simulink model "library"  (R2026b)
settings: Solver=VariableStepAuto
undefined symbols (not defined in the file or in its folder): A_mis_sT, D_b, D_p, D_w, DiscIntNeverNeededParam, fi_acc, fixedStep, k_scale, max_slew_rate, N_B, P_max, P_vec, psi_acc, R_E, sT_bias, theta_acc, Ts
libraries: $bdroot x15, matrix_library x4, simulink x2, backup x1
settings Model: Creator=laythe  LastModifiedBy=laythe

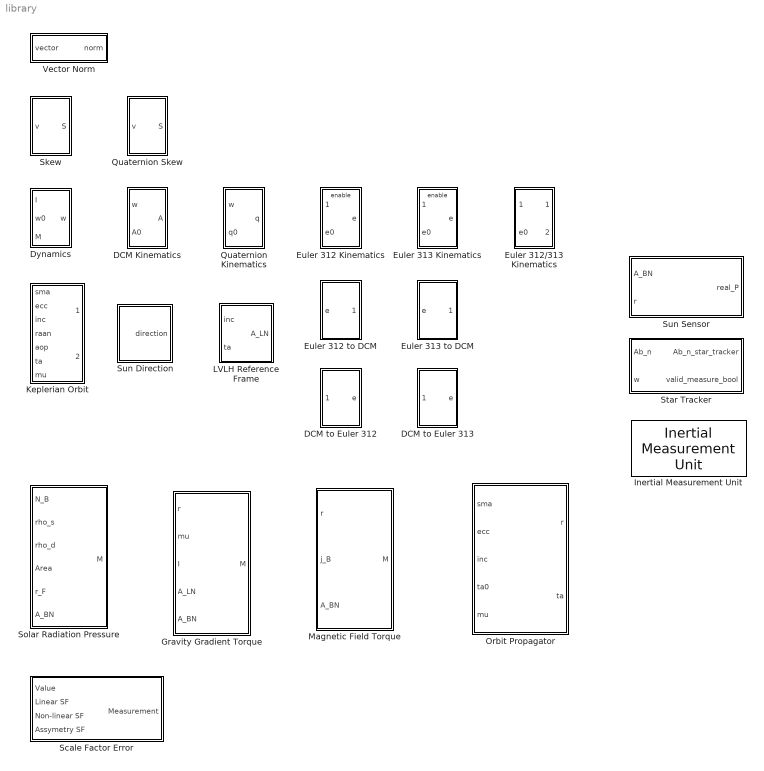
== system library ==
  DCM Kinematics : Subsystem
  DCM to Euler 312 : Subsystem
  DCM to Euler 313 : Subsystem
  Dynamics : Subsystem
  Euler 312 Kinematics : Subsystem
  Euler 312 to DCM : Subsystem
  Euler 312/313 Kinematics : Subsystem
  Euler 313 Kinematics : Subsystem
  Euler 313 to DCM : Subsystem
  Gravity Gradient Torque : Subsystem
  Inertial Measurement Unit : backup/Inertial Measurement Unit  SystemSampleTime=-1  VariantActivationTime=update diagram  EmptyChoice=off  PassThrough=off  PassThroughVariantControl=(default)  EmptyChoiceVariantControl=(default)  AllowFlexibleInterface=on  Latency=0  AutoFrameSizeCalculation=off
  Keplerian Orbit : Subsystem
  LVLH Reference Frame : Subsystem  Description=Inputs: theta_rad (true anomaly), inclination_rad; scalar angles in radians. Output: 3x3 A_LN = Rz_passive(theta)*Rx_passive(i). Maps inertial columns to radial/transverse/normal axes for RAAN=argument of periapsis=0. Exactly the supplied matrix product. No workspace variables.
  Magnetic Field Torque : Subsystem
  Orbit Propagator : Subsystem
  Quaternion Kinematics : Subsystem
  Quaternion Skew : Subsystem
  Scale Factor Error : Subsystem
  Skew : Subsystem
  Solar Radiation Pressure : Subsystem
  Star Tracker : Subsystem
  Sun Direction : Subsystem
  Sun Sensor : Subsystem
  Vector Norm : Subsystem

== system library/DCM Kinematics ==
  w : Inport
  A0 : Inport  Port=2
  Gain : Gain  Gain=-1
  Gain1 : Gain  Gain=1.5
  Gain2 : Gain  Gain=0.5
  Integrator : Integrator  InitialConditionSource=external
  Matrix Multiply : Product  Multiplication=Matrix(*)
  Matrix Multiply1 : Product  Multiplication=Matrix(*)
  Matrix Multiply2 : Product  Multiplication=Matrix(*)
  Skew : $bdroot/Skew  SystemSampleTime=-1  VariantActivationTime=update diagram  EmptyChoice=off  PassThrough=off  PassThroughVariantControl=(default)  EmptyChoiceVariantControl=(default)  AllowFlexibleInterface=on  Latency=0  AutoFrameSizeCalculation=off
  Subtract : Sum  Inputs=+-
  Transpose : Math  Operator=transpose
  A : Outport
  wires:
  Matrix Multiply/1 -> Integrator/1
  A0/1 -> Integrator/2
  Gain/1 -> Matrix Multiply/1
  Skew/1 -> Gain/1
  w/1 -> Skew/1
  Subtract/1 -> Matrix Multiply/2, A/1
  Integrator/1 -> Matrix Multiply2/2, Transpose/1, Matrix Multiply1/1, Gain1/1
  Transpose/1 -> Matrix Multiply1/2
  Matrix Multiply1/1 -> Matrix Multiply2/1
  Matrix Multiply2/1 -> Gain2/1
  Gain1/1 -> Subtract/1
  Gain2/1 -> Subtract/2

== system library/DCM to Euler 312 ==
  DCM : Inport
  Asin : Trigonometry  Operator=asin
  Atan1 : Trigonometry  Operator=atan2
  Atan2 : Trigonometry  Operator=atan2
  Demux : Demux  Outputs=9
  Gain : Gain  Gain=-1
  Gain1 : Gain  Gain=-1
  Mux : Mux  Inputs=3
  Reshape : Reshape  OutputDimensionality=Customize  OutputDimensions=[9,1]
  e : Outport
  wires:
  Demux/8 -> Asin/1
  Asin/1 -> Mux/2
  Atan2/1 -> Mux/1
  Atan1/1 -> Mux/3
  Demux/5 -> Atan2/2
  Demux/9 -> Atan1/2
  Gain/1 -> Atan2/1
  Demux/2 -> Gain/1
  Demux/7 -> Gain1/1
  Gain1/1 -> Atan1/1
  DCM/1 -> Reshape/1
  Reshape/1 -> Demux/1
  Mux/1 -> e/1

== system library/DCM to Euler 313 ==
  DCM : Inport
  Asin : Trigonometry  Operator=acos
  Atan1 : Trigonometry  Operator=atan2
  Atan2 : Trigonometry  Operator=atan2
  Demux : Demux  Outputs=9
  Gain : Gain  Gain=-1
  Mux : Mux  Inputs=3
  Reshape1 : Reshape  OutputDimensionality=Customize  OutputDimensions=[9,1]
  e : Outport
  wires:
  Reshape1/1 -> Demux/1
  Asin/1 -> Mux/2
  Atan2/1 -> Mux/1
  Atan1/1 -> Mux/3
  Gain/1 -> Atan2/2
  Demux/3 -> Atan2/1
  Demux/6 -> Gain/1
  Demux/9 -> Asin/1
  Demux/7 -> Atan1/1
  Demux/8 -> Atan1/2
  Mux/1 -> e/1
  DCM/1 -> Reshape1/1

== system library/Dynamics ==
  I : Inport
  w0 : Inport  Port=2
  M : Inport  Port=3
  Cross Product : matrix_library/Cross Product
  Integrator : Integrator  InitialConditionSource=external
  Matrix Multiply : Product  Multiplication=Matrix(*)
  Matrix Multiply1 : Product  Multiplication=Matrix(*)
  Product : Product  Inputs=/  Multiplication=Matrix(*)
  Sum : Sum  Inputs=|++
  w : Outport
  wires:
  Product/1 -> Matrix Multiply1/1
  Matrix Multiply1/1 -> Integrator/1
  Integrator/1 -> w/1, Matrix Multiply/2, Cross Product/2
  Matrix Multiply/1 -> Cross Product/1
  w0/1 -> Integrator/2
  I/1 -> Product/1, Matrix Multiply/1
  Cross Product/1 -> Sum/1
  Sum/1 -> Matrix Multiply1/2
  M/1 -> Sum/2

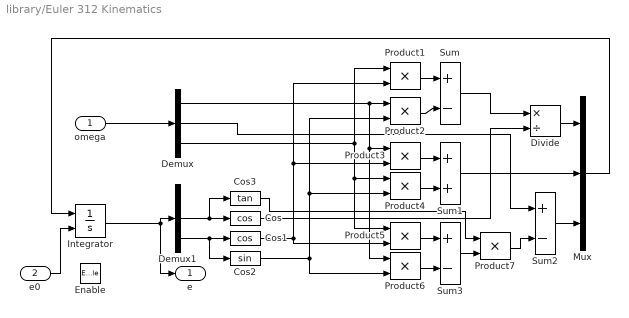
== system library/Euler 312 Kinematics ==
  omega : Inport
  e0 : Inport  Port=2
  Enable : EnablePort  StatesWhenEnabling=reset
  Cos : Trigonometry  Operator=cos
  Cos1 : Trigonometry  Operator=cos
  Cos2 : Trigonometry
  Cos3 : Trigonometry  Operator=tan
  Demux : Demux  Outputs=3
  Demux1 : Demux  Outputs=3
  Divide : Product  Inputs=*/
  Integrator : Integrator  InitialConditionSource=external
  Mux : Mux  Inputs=3
  Product{1..7} (7 alike) : Product
  Sum : Sum  Inputs=+-
  Sum1 : Sum
  Sum2 : Sum  Inputs=+-
  Sum3 : Sum  Inputs=+-
  e : Outport
  wires:
  omega/1 -> Demux/1
  e0/1 -> Integrator/2
  Cos/1 -> Divide/2
  Demux1/2 -> Cos3/1, Cos/1
  Divide/1 -> Mux/1
  Demux1/3 -> Cos2/1, Cos1/1
  Product1/1 -> Sum/1
  Product2/1 -> Sum/2
  Sum/1 -> Divide/1
  Demux/3 -> Product1/1, Product5/1, Product4/1
  Demux/1 -> Product6/1, Product3/1, Product2/1
  Cos1/1 -> Product3/2, Product1/2, Product5/2
  Cos2/1 -> Product6/2, Product4/2, Product2/2
  Product3/1 -> Sum1/1
  Product4/1 -> Sum1/2
  Sum1/1 -> Mux/2
  Sum2/1 -> Mux/3
  Demux/2 -> Sum2/1
  Product5/1 -> Sum3/1
  Product6/1 -> Sum3/2
  Sum3/1 -> Product7/2
  Product7/1 -> Sum2/2
  Cos3/1 -> Product7/1
  Integrator/1 -> Demux1/1, e/1
  Mux/1 -> Integrator/1

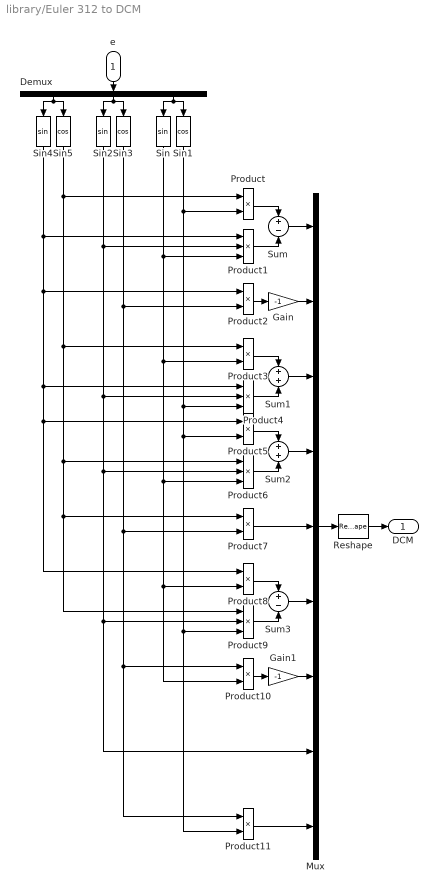
== system library/Euler 312 to DCM ==
  e : Inport
  Demux : Demux  Outputs=3
  Gain : Gain  Gain=-1
  Gain1 : Gain  Gain=-1
  Mux : Mux  Inputs=9
  Product{,2..3,5,7..8,10..11} (8 alike) : Product
  Product{1,4,6,9} (4 alike) : Product  Inputs=3
  Reshape : Reshape  OutputDimensionality=Customize  OutputDimensions=[3,3]
  Sin : Trigonometry
  Sin1 : Trigonometry  Operator=cos
  Sin2 : Trigonometry
  Sin3 : Trigonometry  Operator=cos
  Sin4 : Trigonometry
  Sin5 : Trigonometry  Operator=cos
  Sum : Sum  Inputs=+|-
  Sum1 : Sum  Inputs=+|+
  Sum2 : Sum  Inputs=+|+
  Sum3 : Sum  Inputs=+|-
  DCM : Outport
  wires:
  e/1 -> Demux/1
  Demux/2 -> Sin2/1, Sin3/1
  Product/1 -> Sum/1
  Product1/1 -> Sum/2
  Sum/1 -> Mux/1
  Reshape/1 -> DCM/1
  Mux/1 -> Reshape/1
  Product4/1 -> Sum1/2
  Product3/1 -> Sum1/1
  Sum1/1 -> Mux/3
  Product5/1 -> Sum2/1
  Product6/1 -> Sum2/2
  Sum2/1 -> Mux/4
  Product7/1 -> Mux/5
  Product9/1 -> Sum3/2
  Product8/1 -> Sum3/1
  Sum3/1 -> Mux/6
  Product11/1 -> Mux/9
  Product2/1 -> Gain/1
  Gain/1 -> Mux/2
  Product10/1 -> Gain1/1
  Gain1/1 -> Mux/7
  Demux/1 -> Sin5/1, Sin4/1
  Demux/3 -> Sin1/1, Sin/1
  Sin5/1 -> Product9/1, Product7/1, Product6/1, Product3/1, Product/1
  Sin1/1 -> Product11/2, Product9/3, Product5/2, Product4/3, Product/2
  Sin4/1 -> Product8/1, Product5/1, Product4/1, Product2/1, Product1/1
  Sin2/1 -> Mux/8, Product9/2, Product6/2, Product4/2, Product1/2
  Sin/1 -> Product10/2, Product8/2, Product6/3, Product3/2, Product1/3
  Sin3/1 -> Product11/1, Product10/1, Product7/2, Product2/2

== system library/Euler 312//313 Kinematics ==
  omega : Inport
  e0 : Inport  Port=2
  DCM to Euler : $bdroot/DCM to Euler 313  SystemSampleTime=-1  VariantActivationTime=update diagram  EmptyChoice=off  PassThrough=off  PassThroughVariantControl=(default)  EmptyChoiceVariantControl=(default)  AllowFlexibleInterface=on  Latency=0  AutoFrameSizeCalculation=off
  DCM to Euler 312 : $bdroot/DCM to Euler 312  SystemSampleTime=-1  VariantActivationTime=update diagram  EmptyChoice=off  PassThrough=off  PassThroughVariantControl=(default)  EmptyChoiceVariantControl=(default)  AllowFlexibleInterface=on  Latency=0  AutoFrameSizeCalculation=off
  Euler 312 Kinematics : $bdroot/Euler 312 Kinematics  SystemSampleTime=-1  VariantActivationTime=update diagram  EmptyChoice=off  PassThrough=off  PassThroughVariantControl=(default)  EmptyChoiceVariantControl=(default)  AllowFlexibleInterface=on  Latency=0  AutoFrameSizeCalculation=off
  Euler 312 to DCM2 : $bdroot/Euler 312 to DCM  SystemSampleTime=-1  VariantActivationTime=update diagram  EmptyChoice=off  PassThrough=off  PassThroughVariantControl=(default)  EmptyChoiceVariantControl=(default)  AllowFlexibleInterface=on  Latency=0  AutoFrameSizeCalculation=off
  Euler 313 Kinematics : $bdroot/Euler 313 Kinematics  SystemSampleTime=-1  VariantActivationTime=update diagram  EmptyChoice=off  PassThrough=off  PassThroughVariantControl=(default)  EmptyChoiceVariantControl=(default)  AllowFlexibleInterface=on  Latency=0  AutoFrameSizeCalculation=off
  Euler 313 to DCM1 : $bdroot/Euler 313 to DCM  SystemSampleTime=-1  VariantActivationTime=update diagram  EmptyChoice=off  PassThrough=off  PassThroughVariantControl=(default)  EmptyChoiceVariantControl=(default)  AllowFlexibleInterface=on  Latency=0  AutoFrameSizeCalculation=off
  NOT : Logic  Operator=NOT  IconShape=distinctive  AllPortsSameDT=off  OutDataTypeStr=boolean
  Switch Controller : Subsystem
  Switch1 : Switch  Criteria=u2 ~= 0  SaturateOnIntegerOverflow=off  InputSameDT=off
  A_BN : Outport
  State : Outport  Port=2
  wires:
  DCM to Euler/1 -> Euler 313 Kinematics/2
  NOT/1 -> Euler 313 Kinematics/Enable
  Euler 313 Kinematics/1 -> Euler 313 to DCM1/1
  Euler 312 Kinematics/1 -> Euler 312 to DCM2/1
  Euler 312 to DCM2/1 -> Switch1/1
  e0/1 -> Switch Controller/2(e0)
  Switch Controller/2(DCM) -> DCM to Euler/1, DCM to Euler 312/1
  Switch Controller/1(State) -> NOT/1, Switch1/2, State/1, Euler 312 Kinematics/Enable
  Euler 313 to DCM1/1 -> Switch1/3
  omega/1 -> Switch Controller/3(w), Euler 313 Kinematics/1, Euler 312 Kinematics/1
  Switch1/1 -> Switch Controller/1(A_BN), A_BN/1
  DCM to Euler 312/1 -> Euler 312 Kinematics/2

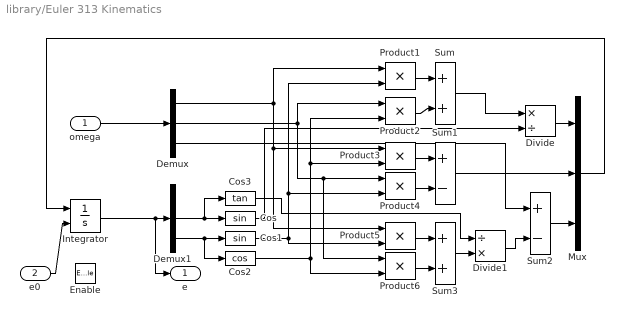
== system library/Euler 313 Kinematics ==
  omega : Inport
  e0 : Inport  Port=2
  Enable : EnablePort  StatesWhenEnabling=reset
  Cos : Trigonometry
  Cos1 : Trigonometry
  Cos2 : Trigonometry  Operator=cos
  Cos3 : Trigonometry  Operator=tan
  Demux : Demux  Outputs=3
  Demux1 : Demux  Outputs=3
  Divide : Product  Inputs=*/
  Divide1 : Product  Inputs=/*
  Integrator : Integrator  InitialConditionSource=external
  Mux : Mux  Inputs=3
  Product{1..6} (6 alike) : Product
  Sum : Sum
  Sum1 : Sum  Inputs=+-
  Sum2 : Sum  Inputs=+-
  Sum3 : Sum
  e : Outport
  wires:
  Mux/1 -> Integrator/1
  Integrator/1 -> e/1, Demux1/1
  Divide1/1 -> Sum2/2
  Sum3/1 -> Divide1/2
  Product6/1 -> Sum3/2
  Product5/1 -> Sum3/1
  Sum2/1 -> Mux/3
  Sum1/1 -> Mux/2
  Product4/1 -> Sum1/2
  Product3/1 -> Sum1/1
  Cos1/1 -> Product4/2, Product1/2, Product5/2
  Demux/1 -> Product1/1, Product5/1, Product3/1
  Sum/1 -> Divide/1
  Product2/1 -> Sum/2
  Product1/1 -> Sum/1
  Demux1/3 -> Cos1/1, Cos2/1
  Divide/1 -> Mux/1
  omega/1 -> Demux/1
  Demux/2 -> Product6/1, Product4/1, Product2/1
  Cos2/1 -> Product6/2, Product3/2, Product2/2
  Demux/3 -> Sum2/1
  e0/1 -> Integrator/2
  Demux1/2 -> Cos3/1, Cos/1
  Cos/1 -> Divide/2
  Cos3/1 -> Divide1/1

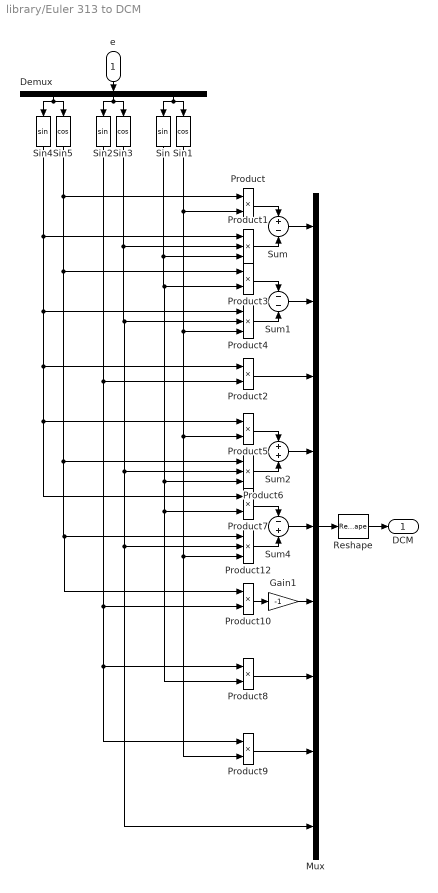
== system library/Euler 313 to DCM ==
  e : Inport
  Demux : Demux  Outputs=3
  Gain1 : Gain  Gain=-1
  Mux : Mux  Inputs=9
  Product{,2..3,5,7..10} (8 alike) : Product
  Product{1,4,6,12} (4 alike) : Product  Inputs=3
  Reshape : Reshape  OutputDimensionality=Customize  OutputDimensions=[3,3]
  Sin : Trigonometry
  Sin1 : Trigonometry  Operator=cos
  Sin2 : Trigonometry
  Sin3 : Trigonometry  Operator=cos
  Sin4 : Trigonometry
  Sin5 : Trigonometry  Operator=cos
  Sum : Sum  Inputs=+|-
  Sum1 : Sum  Inputs=-|-
  Sum2 : Sum  Inputs=+|+
  Sum4 : Sum  Inputs=-|+
  DCM : Outport
  wires:
  e/1 -> Demux/1
  Demux/2 -> Sin2/1, Sin3/1
  Product/1 -> Sum/1
  Product1/1 -> Sum/2
  Sum/1 -> Mux/1
  Reshape/1 -> DCM/1
  Mux/1 -> Reshape/1
  Product5/1 -> Sum2/1
  Product6/1 -> Sum2/2
  Sum2/1 -> Mux/4
  Demux/1 -> Sin5/1, Sin4/1
  Demux/3 -> Sin1/1, Sin/1
  Product4/1 -> Sum1/2
  Sum1/1 -> Mux/2
  Product3/1 -> Sum1/1
  Product2/1 -> Mux/3
  Sum4/1 -> Mux/5
  Product12/1 -> Sum4/2
  Product7/1 -> Sum4/1
  Product10/1 -> Gain1/1
  Gain1/1 -> Mux/6
  Product8/1 -> Mux/7
  Product9/1 -> Mux/8
  Sin5/1 -> Product10/1, Product12/1, Product6/1, Product3/1, Product/1
  Sin1/1 -> Product9/2, Product12/3, Product5/2, Product4/3, Product/2
  Sin4/1 -> Product7/1, Product5/1, Product2/1, Product4/1, Product1/1
  Sin3/1 -> Mux/9, Product12/2, Product6/2, Product4/2, Product1/2
  Sin/1 -> Product8/2, Product7/2, Product6/3, Product3/2, Product1/3
  Sin2/1 -> Product9/1, Product8/1, Product10/2, Product2/2

== system library/Gravity Gradient Torque ==
  r : Inport
  mu : Inport  Port=2
  I : Inport  Port=3
  A_LN : Inport  Port=4
  A_BN : Inport  Port=5
  Constant : Constant  Value=[1 0 0]
  Constant1 : Constant  Value=3
  Cross Product : matrix_library/Cross Product
  Divide : Product  Inputs=*/
  Gain : Gain  Gain=3
  Matrix Multiply : Product  Multiplication=Matrix(*)
  Matrix Multiply1 : Product  Multiplication=Matrix(*)
  Matrix Multiply2 : Product  Multiplication=Matrix(*)
  Power : Math  Operator=pow
  Product2 : Product
  Transpose : Math  Operator=transpose
  Vector Norm : $bdroot/Vector Norm  SystemSampleTime=-1  VariantActivationTime=update diagram  EmptyChoice=off  PassThrough=off  PassThroughVariantControl=(default)  EmptyChoiceVariantControl=(default)  AllowFlexibleInterface=on  Latency=0  AutoFrameSizeCalculation=off
  M : Outport
  wires:
  Matrix Multiply1/1 -> Cross Product/2
  A_LN/1 -> Transpose/1
  Cross Product/1 -> M/1
  Matrix Multiply/1 -> Matrix Multiply2/1
  Constant/1 -> Matrix Multiply2/2
  Transpose/1 -> Matrix Multiply/2
  Product2/1 -> Cross Product/1
  A_BN/1 -> Matrix Multiply/1
  Matrix Multiply2/1 -> Product2/2, Matrix Multiply1/2
  I/1 -> Matrix Multiply1/1
  Divide/1 -> Gain/1
  Gain/1 -> Product2/1
  Power/1 -> Divide/2
  Constant1/1 -> Power/2
  mu/1 -> Divide/1
  r/1 -> Vector Norm/1
  Vector Norm/1 -> Power/1

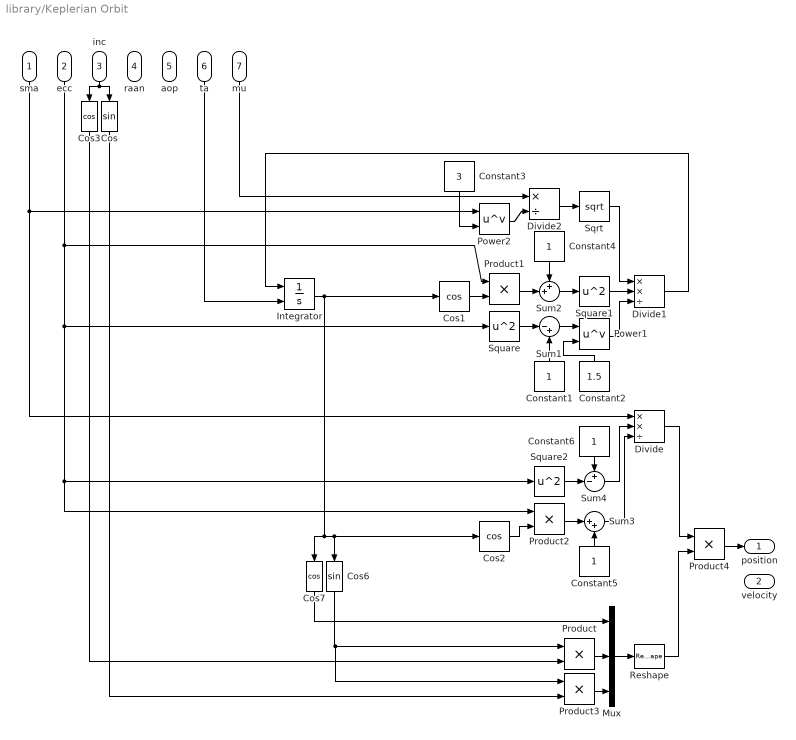
== system library/Keplerian Orbit ==
  sma : Inport
  ecc : Inport  Port=2
  inc : Inport  Port=3
  raan : Inport  Port=4
  aop : Inport  Port=5
  ta : Inport  Port=6
  mu : Inport  Port=7
  Constant{1,4..6} (4 alike) : Constant
  Constant2 : Constant  Value=1.5
  Constant3 : Constant  Value=3
  Cos : Trigonometry
  Cos{1..3,7} (4 alike) : Trigonometry  Operator=cos
  Cos6 : Trigonometry
  Divide : Product  Inputs=**/
  Divide1 : Product  Inputs=**/
  Divide2 : Product  Inputs=*/
  Integrator : Integrator  InitialConditionSource=external
  Mux : Mux  Inputs=3
  Power1 : Math  Operator=pow
  Power2 : Math  Operator=pow
  Product{,1..4} (5 alike) : Product
  Reshape : Reshape  OutputDimensionality=Customize  OutputDimensions=[3,1]
  Sqrt : Sqrt
  Square : Math  Operator=square
  Square1 : Math  Operator=square
  Square2 : Math  Operator=square
  Sum1 : Sum  Inputs=|-+
  Sum2 : Sum  Inputs=++|
  Sum3 : Sum  Inputs=|++
  Sum4 : Sum  Inputs=+-|
  position : Outport
  velocity : Outport  Port=2
  wires:
  ta/1 -> Integrator/2
  ecc/1 -> Product1/1, Product2/1, Square2/1, Square/1
  Integrator/1 -> Cos6/1, Cos2/1, Cos7/1, Cos1/1
  Divide2/1 -> Sqrt/1
  Power2/1 -> Divide2/2
  Constant3/1 -> Power2/2
  sma/1 -> Divide/1, Power2/1
  Sqrt/1 -> Divide1/1
  mu/1 -> Divide2/1
  Square1/1 -> Divide1/2
  Product1/1 -> Sum2/2
  Constant4/1 -> Sum2/1
  Sum2/1 -> Square1/1
  Cos1/1 -> Product1/2
  Square/1 -> Sum1/1
  Sum1/1 -> Power1/1
  Power1/1 -> Divide1/3
  Constant1/1 -> Sum1/2
  Constant2/1 -> Power1/2
  Divide1/1 -> Integrator/1
  Cos2/1 -> Product2/2
  Product2/1 -> Sum3/1
  Constant5/1 -> Sum3/2
  Constant6/1 -> Sum4/1
  Square2/1 -> Sum4/2
  Sum3/1 -> Divide/3
  Sum4/1 -> Divide/2
  inc/1 -> Cos/1, Cos3/1
  Product/1 -> Mux/2
  Product3/1 -> Mux/3
  Cos7/1 -> Mux/1
  Cos6/1 -> Product3/1, Product/1
  Cos3/1 -> Product/2
  Cos/1 -> Product3/2
  Mux/1 -> Reshape/1
  Reshape/1 -> Product4/2
  Divide/1 -> Product4/1
  Product4/1 -> position/1

== system library/LVLH Reference Frame ==
  inc : Inport  PortDimensions=1
  ta : Inport  Port=2  PortDimensions=1
  -sin(inc) : Gain  Gain=-1
  -sin(ta) : Gain  Gain=-1
  Row 1 : Mux  Inputs=3
  Row 2 : Mux  Inputs=3
  Row 3 : Mux  Inputs=3
  assemble_A_LN : Concatenate  NumInputs=3  Mode=Multidimensional array
  cos(ta) * cos(inc) : Product
  cos(ta) * sin(inc) : Product
  inc_sincos : Trigonometry  Operator=sincos
  row1_reshape : Reshape  OutputDimensionality=Row vector (2-D)
  row2_reshape : Reshape  OutputDimensionality=Row vector (2-D)
  row3_reshape : Reshape  OutputDimensionality=Row vector (2-D)
  sin(ta) * cos(inc) : Product
  sin(ta) * sin(inc) : Product
  theta_sincos : Trigonometry  Operator=sincos
  zero : Constant  Value=0
  A_LN : Outport
  wires:
  assemble_A_LN/1 -> A_LN/1
  row3_reshape/1 -> assemble_A_LN/3
  row2_reshape/1 -> assemble_A_LN/2
  row1_reshape/1 -> assemble_A_LN/1
  Row 3/1 -> row3_reshape/1
  -sin(inc)/1 -> Row 3/2
  zero/1 -> Row 3/1
  Row 2/1 -> row2_reshape/1
  cos(ta) * sin(inc)/1 -> Row 2/3
  cos(ta) * cos(inc)/1 -> Row 2/2
  -sin(ta)/1 -> Row 2/1
  Row 1/1 -> row1_reshape/1
  sin(ta) * sin(inc)/1 -> Row 1/3
  sin(ta) * cos(inc)/1 -> Row 1/2
  theta_sincos/2 -> cos(ta) * sin(inc)/1, cos(ta) * cos(inc)/1, Row 1/1
  inc_sincos/2 -> Row 3/3, cos(ta) * cos(inc)/2, sin(ta) * cos(inc)/2
  inc_sincos/1 -> cos(ta) * sin(inc)/2, -sin(inc)/1, sin(ta) * sin(inc)/2
  theta_sincos/1 -> sin(ta) * cos(inc)/1, -sin(ta)/1, sin(ta) * sin(inc)/1
  inc/1 -> inc_sincos/1
  ta/1 -> theta_sincos/1

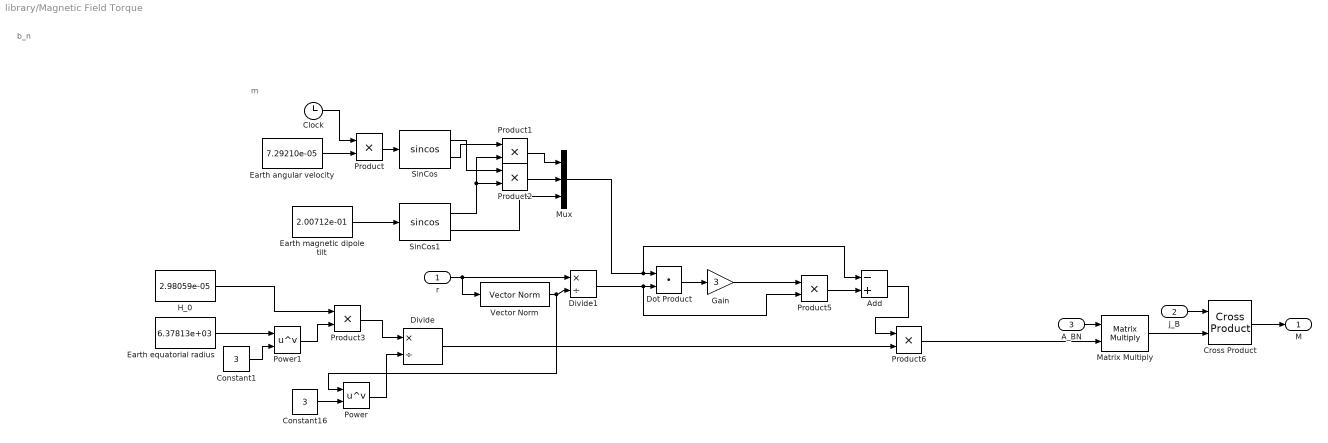
== system library/Magnetic Field Torque ==
  note: b_n
  note: m
  r : Inport
  j_B : Inport  Port=2
  A_BN : Inport  Port=3
  Add : Sum  Inputs=-+
  Clock : Clock
  Constant1 : Constant  Value=3
  Constant16 : Constant  Value=3
  Cross Product : matrix_library/Cross Product
  Divide : Product  Inputs=*/
  Divide1 : Product  Inputs=*/
  Dot Product : DotProduct  OutDataTypeStr=Inherit: Inherit via internal rule
  Earth angular velocity : Constant  Value=7.29210e-05
  Earth equatorial radius : Constant  Value=6.37813e+03
  Earth magnetic dipole tilt : Constant  Value=2.00712e-01
  Gain : Gain  Gain=3
  H_0 : Constant  Value=2.98059e-05
  Matrix Multiply : Product  Multiplication=Matrix(*)
  Mux : Mux  Inputs=3
  Power : Math  Operator=pow
  Power1 : Math  Operator=pow
  Product{,1..3,5..6} (6 alike) : Product
  SinCos : Trigonometry  Operator=sincos
  SinCos1 : Trigonometry  Operator=sincos
  Vector Norm : $bdroot/Vector Norm  SystemSampleTime=-1  VariantActivationTime=update diagram  EmptyChoice=off  PassThrough=off  PassThroughVariantControl=(default)  EmptyChoiceVariantControl=(default)  AllowFlexibleInterface=on  Latency=0  AutoFrameSizeCalculation=off
  M : Outport
  wires:
  Earth equatorial radius/1 -> Power1/1
  Constant16/1 -> Power/2
  Earth magnetic dipole tilt/1 -> SinCos1/1
  Product3/1 -> Divide/1
  Power/1 -> Divide/2
  H_0/1 -> Product3/1
  SinCos1/2 -> Mux/3
  Product5/1 -> Add/2
  SinCos/2 -> Product1/1
  Mux/1 -> Add/1, Dot Product/1
  SinCos1/1 -> Product2/2, Product1/2
  Product2/1 -> Mux/2
  Divide/1 -> Product6/2
  Gain/1 -> Product5/1
  Product1/1 -> Mux/1
  Product/1 -> SinCos/1
  SinCos/1 -> Product2/1
  Cross Product/1 -> M/1
  r/1 -> Vector Norm/1, Divide1/1
  Add/1 -> Product6/1
  A_BN/1 -> Matrix Multiply/1
  Product6/1 -> Matrix Multiply/2
  Matrix Multiply/1 -> Cross Product/2
  Constant1/1 -> Power1/2
  Power1/1 -> Product3/2
  Divide1/1 -> Product5/2, Dot Product/2
  Clock/1 -> Product/1
  Earth angular velocity/1 -> Product/2
  j_B/1 -> Cross Product/1
  Dot Product/1 -> Gain/1
  Vector Norm/1 -> Power/1, Divide1/2

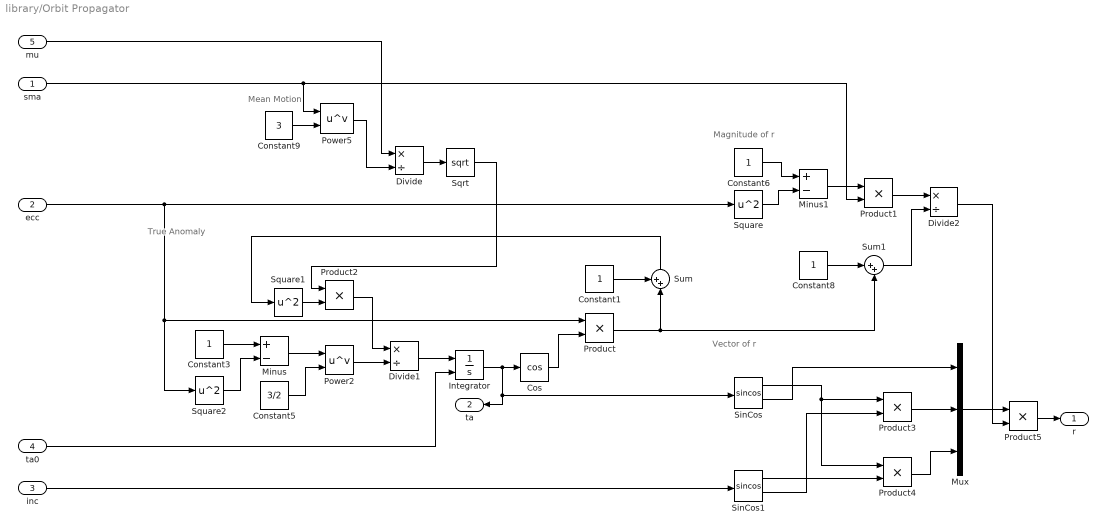
== system library/Orbit Propagator ==
  note: Mean Motion
  note: Vector of r
  note: Magnitude of r
  note: True Anomaly
  sma : Inport
  ecc : Inport  Port=2
  inc : Inport  Port=3
  ta0 : Inport  Port=4
  mu : Inport  Port=5
  Constant{1,3,6,8} (4 alike) : Constant
  Constant5 : Constant  Value=3/2
  Constant9 : Constant  Value=3
  Cos : Trigonometry  Operator=cos
  Divide : Product  Inputs=*/
  Divide1 : Product  Inputs=*/
  Divide2 : Product  Inputs=*/
  Integrator : Integrator  InitialConditionSource=external
  Minus : Sum  Inputs=+-
  Minus1 : Sum  Inputs=+-
  Mux : Mux  Inputs=3
  Power2 : Math  Operator=pow
  Power5 : Math  Operator=pow
  Product{,1..5} (6 alike) : Product
  SinCos : Trigonometry  Operator=sincos
  SinCos1 : Trigonometry  Operator=sincos
  Sqrt : Sqrt
  Square : Math  Operator=square
  Square1 : Math  Operator=square
  Square2 : Math  Operator=square
  Sum : Sum  Inputs=++|
  Sum1 : Sum  Inputs=|++
  r : Outport
  ta : Outport  Port=2
  wires:
  Product5/1 -> r/1
  inc/1 -> SinCos1/1
  Sum1/1 -> Divide2/2
  Product1/1 -> Divide2/1
  Minus1/1 -> Product1/1
  Square/1 -> Minus1/2
  Constant6/1 -> Minus1/1
  Product/1 -> Sum1/2, Sum/2
  Constant1/1 -> Sum/1
  Cos/1 -> Product/2
  Divide2/1 -> Product5/2
  Minus/1 -> Power2/1
  Power2/1 -> Divide1/2
  Square2/1 -> Minus/2
  Integrator/1 -> ta/1, SinCos/1, Cos/1
  Product4/1 -> Mux/3
  ta0/1 -> Integrator/2
  Divide1/1 -> Integrator/1
  SinCos/2 -> Mux/1
  Constant5/1 -> Power2/2
  Constant3/1 -> Minus/1
  ecc/1 -> Square/1, Square2/1, Product/1
  Product3/1 -> Mux/2
  Constant8/1 -> Sum1/1
  sma/1 -> Power5/1, Product1/2
  Mux/1 -> Product5/1
  Square1/1 -> Product2/2
  Product2/1 -> Divide1/1
  mu/1 -> Divide/1
  Sqrt/1 -> Product2/1
  Constant9/1 -> Power5/2
  Power5/1 -> Divide/2
  Divide/1 -> Sqrt/1
  Sum/1 -> Square1/1
  SinCos/1 -> Product4/1, Product3/1
  SinCos1/2 -> Product3/2
  SinCos1/1 -> Product4/2

== system library/Quaternion Kinematics ==
  w : Inport
  q0 : Inport  Port=2
  Gain : Gain  Gain=0.5
  Integrator : Integrator  InitialConditionSource=external
  Matrix Multiply : Product  Multiplication=Matrix(*)
  Quaternion Skew : $bdroot/Quaternion Skew  SystemSampleTime=-1  VariantActivationTime=update diagram  EmptyChoice=off  PassThrough=off  PassThroughVariantControl=(default)  EmptyChoiceVariantControl=(default)  AllowFlexibleInterface=on  Latency=0  AutoFrameSizeCalculation=off
  q : Outport
  wires:
  Matrix Multiply/1 -> Integrator/1
  q0/1 -> Integrator/2
  Gain/1 -> Matrix Multiply/1
  Quaternion Skew/1 -> Gain/1
  w/1 -> Quaternion Skew/1
  Integrator/1 -> Matrix Multiply/2, q/1

== system library/Quaternion Skew ==
  v : Inport
  Constant3 : Constant  Value=0
  Demux : Demux  Outputs=3
  Gain{1..6} (6 alike) : Gain  Gain=-1
  Mux : Mux  Inputs=16
  Reshape : Reshape  OutputDimensionality=Customize  OutputDimensions=[4,4]
  S : Outport
  wires:
  v/1 -> Demux/1
  Constant3/1 -> Mux/1, Mux/11, Mux/16, Mux/6
  Demux/3 -> Gain5/1, Mux/12, Gain6/1, Mux/2
  Gain6/1 -> Mux/5
  Gain1/1 -> Mux/3
  Demux/2 -> Gain2/1, Mux/9, Gain1/1, Mux/8
  Gain2/1 -> Mux/14
  Demux/1 -> Gain4/1, Gain3/1, Mux/7, Mux/4
  Gain3/1 -> Mux/10
  Gain4/1 -> Mux/13
  Gain5/1 -> Mux/15
  Mux/1 -> Reshape/1
  Reshape/1 -> S/1

== system library/Scale Factor Error ==
  Value : Inport
  Linear SF : Inport  Port=2
  Non-linear SF : Inport  Port=3
  Assymetry SF : Inport  Port=4
  Abs : Abs  SaturateOnIntegerOverflow=off
  Product : Product
  Product1 : Product
  Product2 : Product
  Square : Math  Operator=square
  Sum : Sum  Inputs=++++
  Measurement : Outport
  wires:
  Sum/1 -> Measurement/1
  Value/1 -> Abs/1, Square/1, Product/1, Sum/1
  Product/1 -> Sum/2
  Linear SF/1 -> Product/2
  Product1/1 -> Sum/3
  Product2/1 -> Sum/4
  Non-linear SF/1 -> Product1/2
  Assymetry SF/1 -> Product2/2
  Square/1 -> Product1/1
  Abs/1 -> Product2/1

== system library/Skew ==
  v : Inport
  Constant3 : Constant  Value=0
  Demux : Demux  Outputs=3
  Gain2 : Gain  Gain=-1
  Gain3 : Gain  Gain=-1
  Gain4 : Gain  Gain=-1
  Mux : Mux  Inputs=9
  Reshape : Reshape  OutputDimensionality=Customize  OutputDimensions=[3,3]
  S : Outport
  wires:
  Reshape/1 -> S/1
  Demux/2 -> Mux/7, Gain3/1
  Demux/3 -> Mux/2, Gain4/1
  v/1 -> Demux/1
  Constant3/1 -> Mux/9, Mux/5, Mux/1
  Mux/1 -> Reshape/1
  Demux/1 -> Mux/6, Gain2/1
  Gain3/1 -> Mux/3
  Gain4/1 -> Mux/4
  Gain2/1 -> Mux/8

== system library/Solar Radiation Pressure ==
  N_B : Inport
  rho_s : Inport  Port=2
  rho_d : Inport  Port=3
  Area : Inport  Port=4
  r_F : Inport  Port=5
  A_BN : Inport  Port=6
  Reshape : Reshape  OutputDimensionality=Row vector (2-D)
  Reshape1 : Reshape  OutputDimensionality=Row vector (2-D)
  Reshape2 : Reshape  OutputDimensionality=Row vector (2-D)
  Reshape3 : Reshape
  Subsystem : Subsystem
  Sum of Elements : Sum  Inputs=+  CollapseMode=Specified dimension  CollapseDim=2
  M : Outport
  wires:
  N_B/1 -> Subsystem/1(N_B)
  r_F/1 -> Subsystem/5(r_F)
  A_BN/1 -> Subsystem/6(A_BN)
  Subsystem/1(M) -> Sum of Elements/1
  Sum of Elements/1 -> Reshape3/1
  Reshape/1 -> Subsystem/4(Area)
  Area/1 -> Reshape/1
  Reshape1/1 -> Subsystem/3(rho_d)
  Reshape2/1 -> Subsystem/2(rho_s)
  rho_s/1 -> Reshape2/1
  rho_d/1 -> Reshape1/1
  Reshape3/1 -> M/1

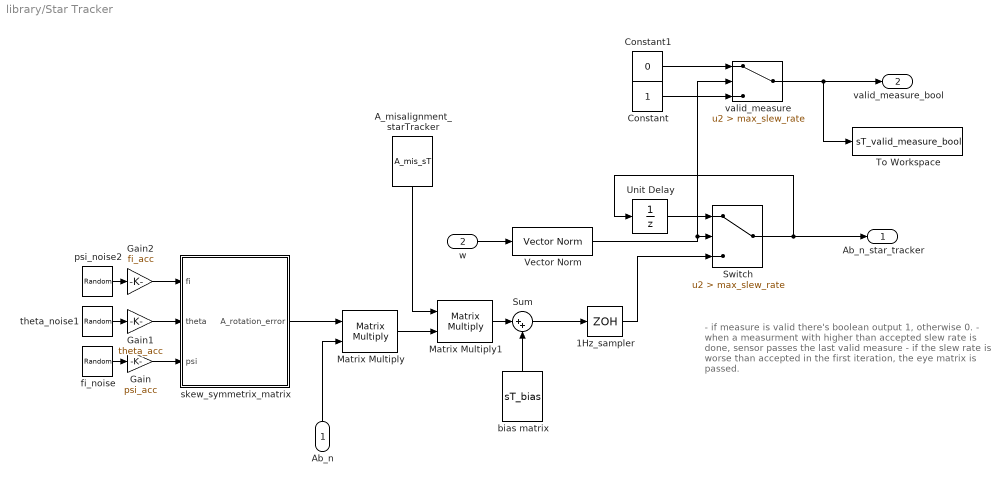
== system library/Star Tracker ==
  note: - if measure is valid there's boolean output 1,
      |  otherwise 0.
      |
      | - when a measurment with higher than accepted
      | slew rate is done, sensor passes the last valid measure
      |
      | - if the slew rate is worse than accepted in the first iteration,
      | the eye matrix is passed.
  Ab_n : Inport
  w : Inport  Port=2
  1Hz_sampler : ZeroOrderHold
  A_misalignment_starTracker : Constant  Value=A_mis_sT
  Constant : Constant
  Constant1 : Constant  Value=0
  Gain : Gain  Gain=psi_acc
  Gain1 : Gain  Gain=theta_acc
  Gain2 : Gain  Gain=fi_acc
  Matrix Multiply : Product  Multiplication=Matrix(*)
  Matrix Multiply1 : Product  Multiplication=Matrix(*)
  Sum : Sum  Inputs=|++
  Switch : Switch  Criteria=u2 > Threshold  Threshold=max_slew_rate  SaturateOnIntegerOverflow=off  InputSameDT=off
  To Workspace : ToWorkspace  VariableName=sT_valid_measure_bool  SaveFormat=Timeseries  SampleTime=-1
  Unit Delay : UnitDelay  InitialCondition=eye(3,3)  SampleTime=-1
  Vector Norm : $bdroot/Vector Norm  SystemSampleTime=-1  VariantActivationTime=update diagram  EmptyChoice=off  PassThrough=off  PassThroughVariantControl=(default)  EmptyChoiceVariantControl=(default)  AllowFlexibleInterface=on  Latency=0  AutoFrameSizeCalculation=off
  bias matrix : Constant  Value=sT_bias
  fi_noise : RandomNumber  Seed=2  SampleTime=0.1
  psi_noise2 : RandomNumber  SampleTime=0.1
  skew_symmetrix_matrix : Subsystem
  theta_noise1 : RandomNumber  Seed=1  SampleTime=0.1
  valid_measure : Switch  Criteria=u2 > Threshold  Threshold=max_slew_rate  SaturateOnIntegerOverflow=off  InputSameDT=off
  Ab_n_star_tracker : Outport
  valid_measure_bool : Outport  Port=2
  wires:
  fi_noise/1 -> Gain/1
  theta_noise1/1 -> Gain1/1
  psi_noise2/1 -> Gain2/1
  Gain1/1 -> skew_symmetrix_matrix/2(theta)
  Gain2/1 -> skew_symmetrix_matrix/1(fi)
  Gain/1 -> skew_symmetrix_matrix/3(psi)
  w/1 -> Vector Norm/1
  Vector Norm/1 -> valid_measure/2, Switch/2
  1Hz_sampler/1 -> Switch/3
  Switch/1 -> Unit Delay/1, Ab_n_star_tracker/1
  Unit Delay/1 -> Switch/1
  valid_measure/1 -> To Workspace/1, valid_measure_bool/1
  Constant/1 -> valid_measure/3
  Constant1/1 -> valid_measure/1
  Matrix Multiply/1 -> Matrix Multiply1/2
  A_misalignment_starTracker/1 -> Matrix Multiply1/1
  Matrix Multiply1/1 -> Sum/1
  Sum/1 -> 1Hz_sampler/1
  bias matrix/1 -> Sum/2
  Ab_n/1 -> Matrix Multiply/2
  skew_symmetrix_matrix/1(A_rotation_error) -> Matrix Multiply/1

== system library/Sun Direction ==
  Clock : Clock
  Constant : Constant  Value=2*pi
  Cos : Trigonometry
  Cos1 : Trigonometry
  Cos2 : Trigonometry  Operator=cos
  Cos3 : Trigonometry  Operator=cos
  Divide : Product  Inputs=*/
  Mux : Mux  Inputs=3
  Product : Product
  Product1 : Product
  Product3 : Product
  Reshape : Reshape  OutputDimensionality=Customize  OutputDimensions=[3,1]
  T : Constant  Value=31558149.76
  epsilon : Constant  Value=0.4091
  direction : Outport
  wires:
  Constant/1 -> Divide/1
  T/1 -> Divide/2
  epsilon/1 -> Cos3/1, Cos/1
  Product/1 -> Mux/2
  Product3/1 -> Mux/3
  Divide/1 -> Product1/1
  Clock/1 -> Product1/2
  Cos3/1 -> Product/2
  Cos/1 -> Product3/2
  Product1/1 -> Cos1/1, Cos2/1
  Cos2/1 -> Mux/1
  Cos1/1 -> Product3/1, Product/1
  Mux/1 -> Reshape/1
  Reshape/1 -> direction/1

== system library/Sun Sensor ==
  A_BN : Inport
  r : Inport  Port=2
  Subsystem : Subsystem
  Sun Direction : $bdroot/Sun Direction  SystemSampleTime=-1  VariantActivationTime=update diagram  EmptyChoice=off  PassThrough=off  PassThroughVariantControl=(default)  EmptyChoiceVariantControl=(default)  AllowFlexibleInterface=on  Latency=0  AutoFrameSizeCalculation=off
  Sun sensor : Subsystem
  real_P : Outport
  wires:
  A_BN/1 -> Sun sensor/1(A_BN)
  Sun Direction/1 -> Sun sensor/3(direction), Subsystem/1(In1)
  Sun sensor/1(real_P) -> real_P/1
  r/1 -> Subsystem/2(r)
  Subsystem/1(eclipse) -> Sun sensor/2(eclipse)

== system library/Vector Norm ==
  vector : Inport
  Dot Product : DotProduct  OutDataTypeStr=Inherit: Inherit via internal rule
  Sqrt : Sqrt
  norm : Outport
  wires:
  Dot Product/1 -> Sqrt/1
  Sqrt/1 -> norm/1
  vector/1 -> Dot Product/2, Dot Product/1

== system library/Euler 312//313 Kinematics/Switch Controller ==
  A_BN : Inport
  e0 : Inport  Port=2
  w : Inport  Port=3
  Abs : Abs  SaturateOnIntegerOverflow=off
  DCM to Euler 312 : $bdroot/DCM to Euler 312  SystemSampleTime=-1  VariantActivationTime=update diagram  EmptyChoice=off  PassThrough=off  PassThroughVariantControl=(default)  EmptyChoiceVariantControl=(default)  AllowFlexibleInterface=on  Latency=0  AutoFrameSizeCalculation=off
  Delay2 : Delay  DelayLength=1  InitialConditionSource=Input port
      settings: InputPortMap=u0,p4
  Euler 312 to DCM3 : $bdroot/Euler 312 to DCM  SystemSampleTime=-1  VariantActivationTime=update diagram  EmptyChoice=off  PassThrough=off  PassThroughVariantControl=(default)  EmptyChoiceVariantControl=(default)  AllowFlexibleInterface=on  Latency=0  AutoFrameSizeCalculation=off
  Relay1 : Relay  OnSwitchValue=deg2rad(80)  OffSwitchValue=deg2rad(75)  OnOutputValue=0  OffOutputValue=1
  Selector_teta1 : Selector  InputPortWidth=3  IndexOptions=Index vector (dialog)  Indices=2  OutputSizes=1  RuntimeRangeChecks=off
  one_step_forward_integrator : Subsystem
  State : Outport
  DCM : Outport  Port=2
  wires:
  Selector_teta1/1 -> Abs/1
  A_BN/1 -> Delay2/1
  Euler 312 to DCM3/1 -> Delay2/2
  DCM to Euler 312/1 -> Selector_teta1/1
  e0/1 -> Euler 312 to DCM3/1
  Abs/1 -> Relay1/1
  Relay1/1 -> State/1
  one_step_forward_integrator/1(DCM_+) -> DCM/1, DCM to Euler 312/1
  Delay2/1 -> one_step_forward_integrator/1(DCM)
  w/1 -> one_step_forward_integrator/2(W)

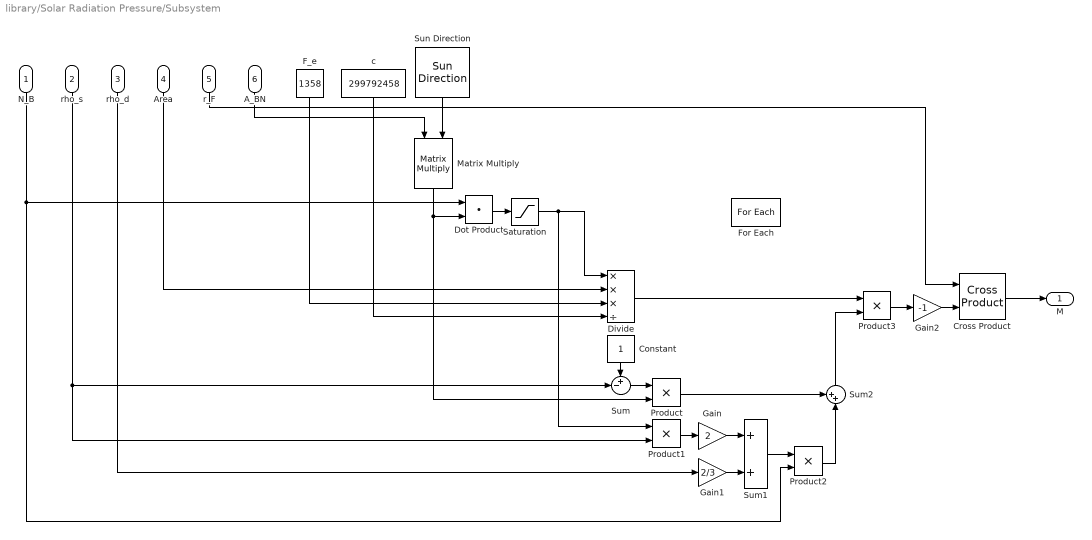
== system library/Solar Radiation Pressure/Subsystem ==
  N_B : Inport  Partition=on  PartitionDimension=2  PartitionWidth=1  PartitionOffset=0
  rho_s : Inport  Port=2  Partition=on  PartitionDimension=2  PartitionWidth=1  PartitionOffset=0
  rho_d : Inport  Port=3  Partition=on  PartitionDimension=2  PartitionWidth=1  PartitionOffset=0
  Area : Inport  Port=4  Partition=on  PartitionDimension=2  PartitionWidth=1  PartitionOffset=0
  r_F : Inport  Port=5  Partition=on  PartitionDimension=2  PartitionWidth=1  PartitionOffset=0
  A_BN : Inport  Port=6
  Constant : Constant
  Cross Product : matrix_library/Cross Product
  Divide : Product  Inputs=***/
  Dot Product : DotProduct  OutDataTypeStr=Inherit: Inherit via internal rule
  F_e : Constant  Value=1358
  For Each : ForEach  DisableCoverage=on
  Gain : Gain  Gain=2
  Gain1 : Gain  Gain=2/3
  Gain2 : Gain  Gain=-1
  Matrix Multiply : Product  Multiplication=Matrix(*)
  Product{,1..3} (4 alike) : Product
  Saturation : Saturate  UpperLimit=1  LowerLimit=0
  Sum : Sum  Inputs=+-|
  Sum1 : Sum
  Sum2 : Sum  Inputs=++|
  Sun Direction : $bdroot/Sun Direction  SystemSampleTime=-1  VariantActivationTime=update diagram  EmptyChoice=off  PassThrough=off  PassThroughVariantControl=(default)  EmptyChoiceVariantControl=(default)  AllowFlexibleInterface=on  Latency=0  AutoFrameSizeCalculation=off
  c : Constant  Value=299792458
  M : Outport  ConcatenationDimension=2
  wires:
  Gain1/1 -> Sum1/2
  rho_d/1 -> Gain1/1
  Product1/1 -> Gain/1
  Product3/1 -> Gain2/1
  Sum/1 -> Product/1
  Product2/1 -> Sum2/2
  Product/1 -> Sum2/1
  N_B/1 -> Product2/2, Dot Product/1
  Gain/1 -> Sum1/1
  rho_s/1 -> Product1/2, Sum/2
  Constant/1 -> Sum/1
  r_F/1 -> Cross Product/1
  Saturation/1 -> Product1/1, Divide/1
  c/1 -> Divide/4
  Matrix Multiply/1 -> Product/2, Dot Product/2
  Divide/1 -> Product3/1
  Cross Product/1 -> M/1
  Sum1/1 -> Product2/1
  Dot Product/1 -> Saturation/1
  Gain2/1 -> Cross Product/2
  Sun Direction/1 -> Matrix Multiply/2
  F_e/1 -> Divide/3
  Area/1 -> Divide/2
  Sum2/1 -> Product3/2
  A_BN/1 -> Matrix Multiply/1

== system library/Star Tracker/skew_symmetrix_matrix ==
  fi : Inport
  theta : Inport  Port=2
  psi : Inport  Port=3
  Constant : Constant
  Gain : Gain  Gain=-1
  Gain1 : Gain  Gain=-1
  Gain2 : Gain  Gain=-1
  Matrix Concatenate : Concatenate  NumInputs=3  Mode=Multidimensional array  ConcatenateDimension=2
  first column : Mux  Inputs=3
  second column : Mux  Inputs=3
  third colum : Mux  Inputs=3
  A_rotation_error : Outport
  wires:
  Matrix Concatenate/1 -> A_rotation_error/1
  Constant/1 -> first column/1, second column/2, third colum/3
  Gain/1 -> first column/2
  fi/1 -> Gain/1, second column/1
  psi/1 -> first column/3, Gain2/1
  Gain1/1 -> second column/3
  theta/1 -> Gain1/1, third colum/2
  Gain2/1 -> third colum/1
  first column/1 -> Matrix Concatenate/1
  second column/1 -> Matrix Concatenate/2
  third colum/1 -> Matrix Concatenate/3

== system library/Sun Sensor/Subsystem ==
  In1 : Inport
  r : Inport  Port=2
  AND : Logic  IconShape=distinctive  AllPortsSameDT=off  OutDataTypeStr=boolean
  Compare To Constant : simulink/Logic and Bit Operations/Compare To Constant  relop=<  const=0  OutDataTypeStr=boolean
  Compare To Constant1 : simulink/Logic and Bit Operations/Compare To Constant  relop=<  const=R_E  OutDataTypeStr=boolean
  Data Type Conversion : DataTypeConversion  OutDataTypeStr=double  SaturateOnIntegerOverflow=off  RndMeth=Floor
  Dot Product : DotProduct  OutDataTypeStr=Inherit: Inherit via internal rule
  Dot Product1 : DotProduct  OutDataTypeStr=Inherit: Inherit via internal rule
  NOT : Logic  Operator=NOT  IconShape=distinctive  AllPortsSameDT=off  OutDataTypeStr=boolean
  Product : Product
  Scope : Scope
      settings: ActiveDisplayYMinimum=-0.12499999999999997  ActiveDisplayYMaximum=1.125  DataLoggingVariableName=ScopeData7
  Sqrt : Sqrt
  r_perp : Sum  Inputs=+-
  eclipse : Outport
  wires:
  Data Type Conversion/1 -> eclipse/1
  AND/1 -> NOT/1, Scope/1
  Dot Product1/1 -> Sqrt/1
  NOT/1 -> Data Type Conversion/1
  Sqrt/1 -> Compare To Constant1/1
  Product/1 -> r_perp/2
  Compare To Constant/1 -> AND/1
  r/1 -> r_perp/1, Dot Product/1
  In1/1 -> Product/2, Dot Product/2
  r_perp/1 -> Dot Product1/1, Dot Product1/2
  Compare To Constant1/1 -> AND/2
  Dot Product/1 -> Product/1, Compare To Constant/1

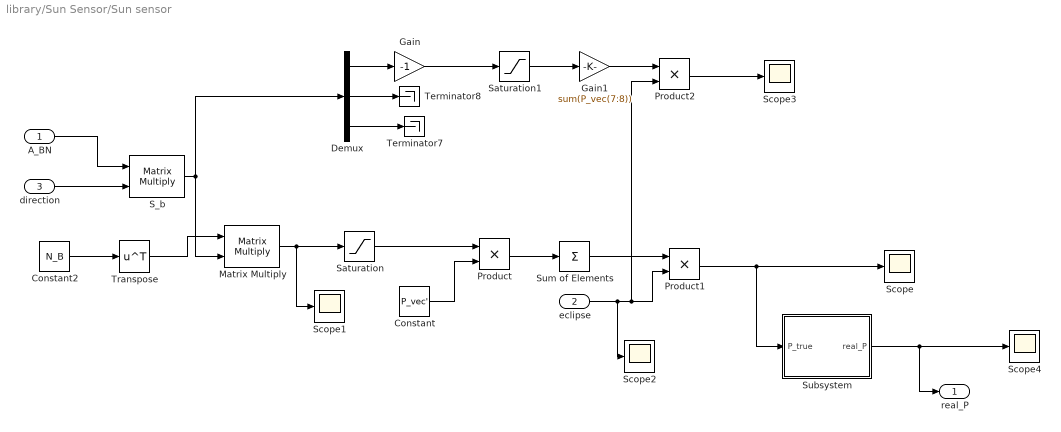
== system library/Sun Sensor/Sun sensor ==
  A_BN : Inport
  eclipse : Inport  Port=2
  direction : Inport  Port=3
  Constant : Constant  Value=P_vec'
  Constant2 : Constant  Value=N_B
  Demux : Demux  Outputs=3
  Gain : Gain  Gain=-1
  Gain1 : Gain  Gain=sum(P_vec(7:8))
  Matrix Multiply : Product  Multiplication=Matrix(*)
  Product : Product
  Product1 : Product
  Product2 : Product
  S_b : Product  Multiplication=Matrix(*)
  Saturation : Saturate  UpperLimit=1  LowerLimit=0
  Saturation1 : Saturate  UpperLimit=1  LowerLimit=0
  Scope{,1..4} (5 alike) : Scope
      Scope settings: ActiveDisplayYMinimum=-0.62909362598000107  ActiveDisplayYMaximum=5.6618426338200107  DataLoggingVariableName=ScopeData9
      Scope1 settings: ActiveDisplayYMinimum=-1.2499296718920987  ActiveDisplayYMaximum=1.2499296718920987  DataLoggingVariableName=ScopeData10
      Scope2 settings: ActiveDisplayYMinimum=-0.12499999999999997  ActiveDisplayYMaximum=1.125  DataLoggingVariableName=ScopeData11
      Scope3 settings: ActiveDisplayYMinimum=-0.62909362598000107  ActiveDisplayYMaximum=5.6618426338200107  DataLoggingVariableName=ScopeData12
      Scope4 settings: ActiveDisplayYMinimum=-2.1294246544747728  ActiveDisplayYMaximum=7.8320158438971825  DataLoggingVariableName=ScopeData13
  Subsystem : Subsystem
  Sum of Elements : Sum  Inputs=+
  Terminator7 : Terminator
  Terminator8 : Terminator
  Transpose : Math  Operator=transpose
  real_P : Outport
  wires:
  A_BN/1 -> S_b/1
  S_b/1 -> Matrix Multiply/2, Demux/1
  direction/1 -> S_b/2
  Matrix Multiply/1 -> Scope1/1, Saturation/1
  Saturation/1 -> Product/1
  Product/1 -> Sum of Elements/1
  Sum of Elements/1 -> Product1/1
  eclipse/1 -> Scope2/1, Product2/2, Product1/2
  Product1/1 -> Subsystem/1(P_true), Scope/1
  Constant/1 -> Product/2
  Constant2/1 -> Transpose/1
  Transpose/1 -> Matrix Multiply/1
  Demux/3 -> Terminator7/1
  Demux/2 -> Terminator8/1
  Demux/1 -> Gain/1
  Gain/1 -> Saturation1/1
  Saturation1/1 -> Gain1/1
  Gain1/1 -> Product2/1
  Product2/1 -> Scope3/1
  Subsystem/1(real_P) -> real_P/1, Scope4/1

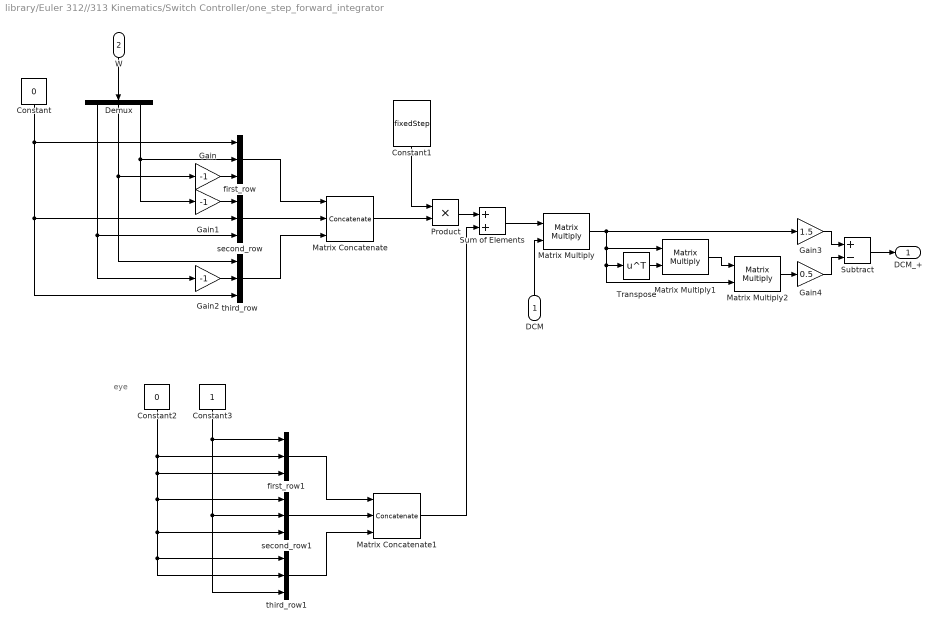
== system library/Euler 312//313 Kinematics/Switch Controller/one_step_forward_integrator ==
  note: eye
  DCM : Inport
  W : Inport  Port=2
  Constant : Constant  Value=0
  Constant1 : Constant  Value=fixedStep
  Constant2 : Constant  Value=0
  Constant3 : Constant
  Demux : Demux  Outputs=3
  Gain : Gain  Gain=-1
  Gain1 : Gain  Gain=-1
  Gain2 : Gain  Gain=-1
  Gain3 : Gain  Gain=1.5
  Gain4 : Gain  Gain=0.5
  Matrix Concatenate : Concatenate  NumInputs=3  Mode=Multidimensional array  ConcatenateDimension=2
  Matrix Concatenate1 : Concatenate  NumInputs=3  Mode=Multidimensional array  ConcatenateDimension=2
  Matrix Multiply : Product  Multiplication=Matrix(*)
  Matrix Multiply1 : Product  Multiplication=Matrix(*)
  Matrix Multiply2 : Product  Multiplication=Matrix(*)
  Product : Product
  Subtract : Sum  Inputs=+-
  Sum of Elements : Sum
  Transpose : Math  Operator=transpose
  first_row : Mux  Inputs=3
  first_row1 : Mux  Inputs=3
  second_row : Mux  Inputs=3
  second_row1 : Mux  Inputs=3
  third_row : Mux  Inputs=3
  third_row1 : Mux  Inputs=3
  DCM_+ : Outport
  wires:
  Subtract/1 -> DCM_+/1
  Matrix Multiply/1 -> Gain3/1, Matrix Multiply1/1, Transpose/1, Matrix Multiply2/2
  Gain3/1 -> Subtract/1
  Transpose/1 -> Matrix Multiply1/2
  Matrix Multiply2/1 -> Gain4/1
  Matrix Multiply1/1 -> Matrix Multiply2/1
  Gain4/1 -> Subtract/2
  third_row/1 -> Matrix Concatenate/3
  second_row/1 -> Matrix Concatenate/2
  first_row/1 -> Matrix Concatenate/1
  Constant/1 -> first_row/1, second_row/2, third_row/3
  Demux/3 -> first_row/2, Gain1/1
  Gain/1 -> first_row/3
  Demux/2 -> third_row/1, Gain/1
  Gain1/1 -> second_row/1
  Demux/1 -> Gain2/1, second_row/3
  DCM/1 -> Matrix Multiply/2
  Constant1/1 -> Product/1
  W/1 -> Demux/1
  Matrix Concatenate/1 -> Product/2
  Product/1 -> Sum of Elements/1
  Sum of Elements/1 -> Matrix Multiply/1
  first_row1/1 -> Matrix Concatenate1/1
  second_row1/1 -> Matrix Concatenate1/2
  third_row1/1 -> Matrix Concatenate1/3
  Constant3/1 -> first_row1/1, third_row1/3, second_row1/2
  Constant2/1 -> first_row1/2, first_row1/3, second_row1/1, third_row1/2, third_row1/1, second_row1/3
  Matrix Concatenate1/1 -> Sum of Elements/2
  Gain2/1 -> third_row/2

== system library/Sun Sensor/Sun sensor/Subsystem ==
  P_true : Inport
  Bias : Constant  Value=D_p/sqrt(2*Ts)
  Mux : Mux  Inputs=2
  Saturation : Saturate  UpperLimit=P_max  LowerLimit=0
  Scope : Scope
      settings: ActiveDisplayYMinimum=-0.12794674810584095  ActiveDisplayYMaximum=3.2352249163905733  DataLoggingVariableName=ScopeData15
  Subsystem : Subsystem
  Sum : Sum  Inputs=+++
  Zero-Order Hold : ZeroOrderHold  SampleTime=0.1
  scale : Gain  Gain=1+k_scale
  real_P : Outport
  wires:
  P_true/1 -> Mux/1, scale/1
  scale/1 -> Mux/2, Sum/1
  Subsystem/1(Noise) -> Sum/3
  Sum/1 -> Saturation/1
  Bias/1 -> Sum/2
  Mux/1 -> Scope/1
  Saturation/1 -> Zero-Order Hold/1
  Zero-Order Hold/1 -> real_P/1

== system library/Sun Sensor/Sun sensor/Subsystem/Subsystem ==
  Discrete Transfer Fcn : DiscreteTransferFcn  Numerator=[0.2696]  Denominator=[1 -0.7304]
  Discrete-Time Integrator : DiscreteIntegrator  SampleTime=0.1  ICPrevOutput=DiscIntNeverNeededParam  ICPrevScaledInput=DiscIntNeverNeededParam
  Gain : Gain  Gain=D_w/sqrt(2*Ts)
  Gain1 : Gain  Gain=D_p/sqrt(2*Ts)
  Gain3 : Gain  Gain=D_b/sqrt(2*Ts)
  Mux : Mux  Inputs=3
  Random Number : RandomNumber  Seed=1  SampleTime=Ts
  Random Number1 : RandomNumber  SampleTime=0.1
  Random Number2 : RandomNumber  SampleTime=0.1
  Scope : Scope
      settings: ActiveDisplayYMinimum=-1.0654992152689575  ActiveDisplayYMaximum=0.96833844465150587  DataLoggingVariableName=ScopeData14
  Sum : Sum  Inputs=+++
  Noise : Outport
  wires:
  Discrete-Time Integrator/1 -> Mux/3
  Sum/1 -> Noise/1
  Gain/1 -> Mux/1, Sum/1
  Random Number/1 -> Gain/1
  Random Number2/1 -> Gain3/1
  Gain3/1 -> Discrete-Time Integrator/1
  Discrete Transfer Fcn/1 -> Mux/2
  Random Number1/1 -> Gain1/1
  Gain1/1 -> Discrete Transfer Fcn/1
  Mux/1 -> Scope/1
